simulink model "EncoderRead"  (R2020b)
settings: Solver=FixedStepAuto  StartTime=0.0  StopTime=1.5  FixedStep=0.0001  RelTol=1e-3
values from neighbouring files (symbols this model uses):
  T = x(3)    [PT1T.m]    (also in SystemID_Setup.m = 0.0001; squarefit_motor.mat = 0.0001)
undefined symbols (not defined in the file or in its folder): National_Instruments, PCIe
libraries: sldrtlib x3, mcbpositiondecoderlib x1
settings Model: SimulationMode=external  ExtModeTrigDuration=100001  Creator=EAL  LastModifiedBy=EAL
settings RTWCC: Description=Simulink Desktop Real-Time  SystemTargetFile=sldrt.tlc  TemplateMakefile=sldrt.tmf  RTWCompilerOptimization=on
settings CodeAppCC: MaxIdLength=95
settings SimulinkDesktopRealTimeCC: TargetPreCompLibLocation=C:\Program Files\MATLAB\R2020b\toolbox\sldrt\lib\win64

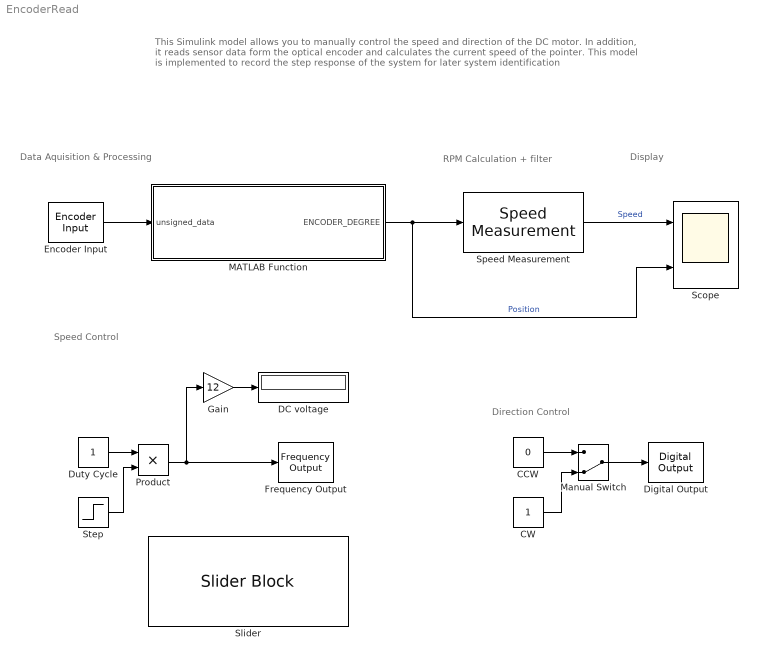
== system EncoderRead ==
  note: This Simulink model allows you to manually control the speed and direction of the DC motor.
      | In addition, it reads sensor data form the optical encoder and calculates the current speed of the pointer.
      |
      | This model is implemented to record the step response of the system for later system identification
  note: Display
  note: RPM Calculation + filter
  note: Data Aquisition & Processing
  note: Speed Control
  note: Direction Control
  CCW : Constant  Value=0  OutDataTypeStr=single
  CW : Constant  OutDataTypeStr=single
  DC voltage : Display
  Digital Output : sldrtlib/Digital Output  SampleTime=0.0001  MaxMissedTicks=10000  ShowMissedTicks=off  YieldWhenWaiting=off  DrvName=National_Instruments/PCIe-6321  DrvAddress=4294967295  DrvOptions=[0 1 0 2 3 0 0]  Channels=1  BitMode=1  InitialValue=0  FinalValue=0
      settings: AttributesFormatString=National Instruments\nPCIe-6321 [auto]  SourceProductBaseCode=WT
  Duty Cycle : Constant  OutMin=[0]  OutMax=[1]  OutDataTypeStr=double
  Encoder Input : sldrtlib/Encoder Input  SampleTime=T  MaxMissedTicks=10000  ShowMissedTicks=off  YieldWhenWaiting=off  DrvName=National_Instruments/PCIe-6321  DrvAddress=4294967295  DrvOptions=[0 1 0 2 3 0 0]  Channels=1  QuadMode=3  IndexPulse=1  InputFilter=Inf  DataType=1
      settings: AttributesFormatString=National Instruments\nPCIe-6321 [auto]
  Frequency Output : sldrtlib/Frequency Output  SampleTime=0.0001  MaxMissedTicks=100000  ShowMissedTicks=off  YieldWhenWaiting=off  DrvName=National_Instruments/PCIe-6321  DrvAddress=4294967295  DrvOptions=[0 1 0 2 3 0 0]  Channels=2  FrequencySource=1  Frequency=15000  FrequencyFinalValue=[]  DutySource=2  Duty=0  DutyFinalValue=0
      settings: AttributesFormatString=National Instruments\nPCIe-6321 [auto]  SourceProductBaseCode=WT
  Gain : Gain  Gain=12
  MATLAB Function : MATLAB Function  TreatAsAtomicUnit=on
  Manual Switch : ManualSwitch  CurrentSetting=0
  Product : Product
  Scope : Scope  NumInputPorts=2
  Slider : SliderBlock  ScaleMax=1
  Speed Measurement : mcbpositiondecoderlib/Speed Measurement  PositionUnit=Degrees  SpeedCalculationMode=Time interval for speed calculation  SampleTimeAsync=T  MaximumApplicationSpeed=1000  SpeedResolution=0.18  DelayLength=300  MaximumMeasurableSpeed=999  MeasurableSpeedResolution=4.6566e-07  SpeedUnit=RPM  PerUnitSpeed=1000  SpeedDataType=double
      settings: SourceProductBaseCode=MT
  Step : Step  Time=0  SampleTime=0
  wires:
  Duty Cycle/1 -> Product/1
  CCW/1 -> Manual Switch/1
  Manual Switch/1 -> Digital Output/1
  CW/1 -> Manual Switch/2
  Gain/1 -> DC voltage/1
  Product/1 -> Frequency Output/1, Gain/1
  Step/1 -> Product/2
  Encoder Input/1 -> MATLAB Function/1(unsigned_data)
  Speed Measurement/1 -> Scope/1  "Speed"
  MATLAB Function/1(ENCODER_DEGREE) -> Speed Measurement/1, Scope/2  "Position"

== matlab function EncoderRead/MATLAB Function ==
  data: unsigned_data input; ENCODER_DEGREE output
function ENCODER_DEGREE = PPR2DEG(unsigned_data)
    ENCODER_PPR = 2000;
    COUNTER_N_BITS = 32;
    THRESHOLD = 2^(COUNTER_N_BITS - 1);
    if (unsigned_data > THRESHOLD)
        ENCODER_DEGREE = (unsigned_data - 2^COUNTER_N_BITS) * 360/ENCODER_PPR;
    else
        ENCODER_DEGREE = unsigned_data * 360/ENCODER_PPR;
    end

end
